simulink model "dc_motor_position_control"  (R2026a)
settings: Solver=VariableStepAuto  StopTime=20  MaxStep=0.01
InitFcn:
  | init_motor;
undefined symbols (not defined in the file or in its folder): ctrl, motor, sensor
libraries: slpidlib x1, simulink x1
settings Model: Creator=seman  LastModifiedBy=seman

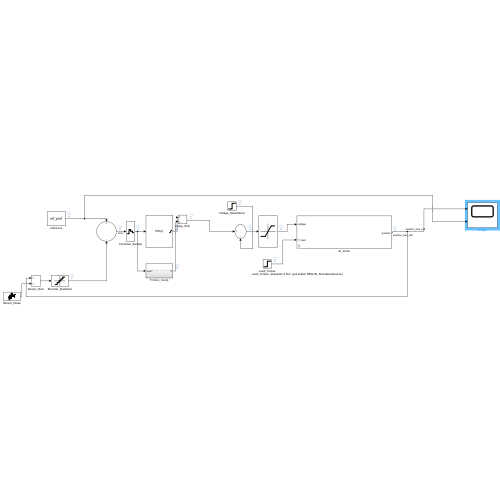
[thumbnail: Simulink's stored preview of the top-level diagram]
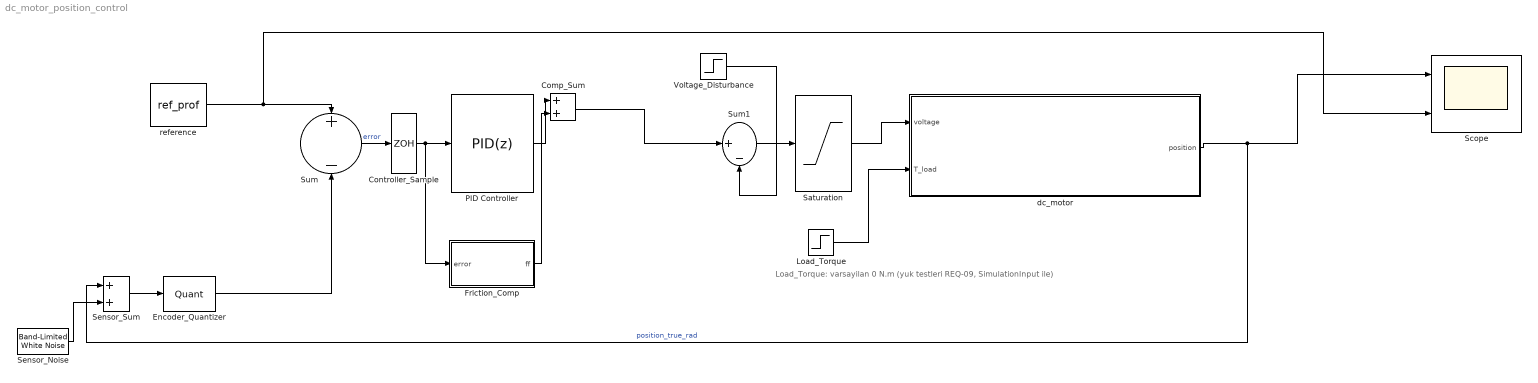
== system dc_motor_position_control ==
  note: Load_Torque: varsayilan 0 N.m (yuk testleri REQ-09, SimulationInput ile)
  Comp_Sum : Sum
  Controller_Sample : ZeroOrderHold  SampleTime=ctrl.Ts
  Encoder_Quantizer : Quantizer  QuantizationInterval=sensor.q_enc
  Friction_Comp : Subsystem
  Load_Torque : Step  Description=Yuk torku girisi (N.m). Varsayilan 0. REQ-09 testleri (run_load_torque_test, run_load_worstcase) basamak yuku SimulationInput ile yalnizca o kosu icin verir.  Time=10  FinalValue=5  SampleTime=0
  PID Controller : slpidlib/PID Controller  Controller=PID  Form=Parallel  TimeDomain=Discrete-time  UseExternalTs=off  SampleTime=ctrl.Ts  IntegratorMethod=Forward Euler  FilterMethod=Backward Euler  ControllerParametersSource=internal  P=ctrl.Kp  I=ctrl.Ki  UseKiTs=off  D=ctrl.Kd  UseExternalDerivativeSource=off  N=ctrl.N  UseFilter=on  TunerSelectOption=Transfer Function Based (PID Tuner App)  InitialConditionSource=internal  InitialConditionForIntegrator=0  InitialConditionForFilter=0  DifferentiatorICPrevScaledInput=0  ExternalReset=none  TrackingMode=off  Kt=1  LimitOutput=on  SatLimitsSource=internal  UpperSaturationLimit=ctrl.Vmax  LowerSaturationLimit=-ctrl.Vmax  LinearizeAsGain=on  AntiWindupMode=back-calculation  Kb=1  LimitIntegrator=off  UpperIntegratorSaturationLimit=inf  LowerIntegratorSaturationLimit=-inf  POutMin=[]  POutMax=[]  IOutMin=[]  IOutMax=[]  DOutMin=[]  DOutMax=[]  NOutMin=[]  NOutMax=[]  SumOutMin=[]  SumOutMax=[]  SaturationOutMin=[]  SaturationOutMax=[]  PParamMin=[]  PParamMax=[]  IParamMin=[]  IParamMax=[]  DParamMin=[]  DParamMax=[]  NParamMin=[]  NParamMax=[]  KbParamMin=[]  KbParamMax=[]  KtParamMin=[]  KtParamMax=[]  KbOutMin=[]  KbOutMax=[]  KtOutMin=[]  KtOutMax=[]  IntegratorOutMin=[]  IntegratorOutMax=[]  FilterOutMin=[]  FilterOutMax=[]  SumI1OutMin=[]  SumI1OutMax=[]  SumI2OutMin=[]  SumI2OutMax=[]  SumI3OutMin=[]  SumI3OutMax=[]  SumI4OutMin=[]  SumI4OutMax=[]  SumDOutMin=[]  SumDOutMax=[]  DifferentiatorOutMin=[]  DifferentiatorOutMax=[]  FilterDiffOutCoefMin=[]  FilterDiffOutCoefMax=[]  ReciprocalOutMin=[]  ReciprocalOutMax=[]  SumDenOutMin=[]  SumDenOutMax=[]  SumNumOutMin=[]  SumNumOutMax=[]  DivideOutMin=[]  DivideOutMax=[]  UdiffTsProdOutMin=[]  UdiffTsProdOutMax=[]  NTsProdOutMin=[]  NTsProdOutMax=[]  UintegralTsProdOutMin=[]  UintegralTsProdOutMax=[]  UngainTsProdOutMin=[]  UngainTsProdOutMax=[]  ClampingZeroOutDataTypeStr=Inherit: Inherit via back propagation  ClampingZeroOutMin=[]  ClampingZeroOutMax=[]  FilterDenConstantOutDataTypeStr=Inherit: Inherit via back propagation  FilterDenConstantOutMin=[]  FilterDenConstantOutMax=[]  PCopyOutDataTypeStr=Inherit: Inherit via back propagation  PCopyOutMin=[]  PCopyOutMax=[]  NCopyOutDataTypeStr=Inherit: Inherit via back propagation  NCopyOutMin=[]  NCopyOutMax=[]  IntegratorContinuousStateAttributes=''  IntegratorStateMustResolveToSignalObject=off  IntegratorRTWStateStorageClass=Auto  FilterContinuousStateAttributes=''  FilterStateMustResolveToSignalObject=off  FilterRTWStateStorageClass=Auto  ParallelPVariant=InternalParameters  IdealPVariant=Disabled  IVariant=InternalParameters  DVariant=InternalParameters  IntegratorVariant=Discrete  SatVariant=Enabled  AWVariant=BackCalculation  PCopyVariant=Disabled  TRVariant=Disabled  FdbkBlocksVariant=Forward  IdealPFdbkVariant=Disabled  SatFdbkVariant=Disabled  DerivativeFilterVariant=BackwardEulerFilter  NVariant=InternalParameters  NCopyVariant=InternalParameters  FilterICVariant=InternalICsFilter  IntegratorICVariant=InternalICs  ExternalResetVariant=Disabled  TRSumVariant=Passthrough  SumFdbkVariant=Disabled  SumVariant=Sum_PID  TsampFilterVariant=InternalTs  TsampNgainVariant=Passthrough  TsampIntegralVariant=Disabled_SignalSpec  ExternalSaturationOutDataTypeStr=Inherit: Same as second input  DerivativeSourceVariant=ErrorSignal  PreIntVariant=InternalPreInt
  Saturation : Saturate  UpperLimit=ctrl.Vmax  LowerLimit=-ctrl.Vmax
  Scope : Scope  NumInputPorts=2
      settings: ActiveDisplayYMinimum=-11.339350762490124  ActiveDisplayYMaximum=102.05415686241113
  Sensor_Noise : simulink/Sources/Band-Limited White Noise  Cov=sensor.noise_cov  Ts=sensor.noise_Ts  seed=[sensor.seed]
  Sensor_Sum : Sum
  Sum : Sum  Inputs=+-
  Sum1 : Sum  Inputs=|+-
  Voltage_Disturbance : Step  Description=Voltaj bozucusu (V). Normalde 0; run_disturbance_test ve run_disturbance_sweep acar.  Time=10  FinalValue=0  SampleTime=0
  dc_motor : Subsystem  InitFcn=""  mask{J=motor.J, B=motor.B, KT=motor.KT, R=motor.R, L=motor.L, KB=motor.KB, Tc=motor.Tc, w_eps=motor.w_eps}
      mask prompts: J "J(KG*M^2)"; B "B(Nm/rad)"; KT "NM/AMPER"; R "R(OHM)"; L "L(H)"; KB "KB(VS/rad)"; Tc "Coulomb surtunme torku (N.m)"; w_eps "Coulomb yumusatma hizi (rad/s)"
  reference : FromWorkspace  Description=Konum referansi (rad). Veri: ref_prof = [zaman konum], init_motor.m icinde. Varsayilan: sabit 50 rad.  VariableName=ref_prof  OutputAfterFinalValue=Holding final value
  wires:
  dc_motor/1(position) -> Scope/1, Sensor_Sum/1  "position_true_rad"
  reference/1 -> Scope/2, Sum/1
  Saturation/1 -> dc_motor/1(voltage)
  Voltage_Disturbance/1 -> Sum1/2
  Sum1/1 -> Saturation/1
  Sensor_Noise/1 -> Sensor_Sum/2
  Sensor_Sum/1 -> Encoder_Quantizer/1
  Encoder_Quantizer/1 -> Sum/2
  Load_Torque/1 -> dc_motor/2(T_load)
  PID Controller/1 -> Comp_Sum/1
  Comp_Sum/1 -> Sum1/1
  Friction_Comp/1(ff) -> Comp_Sum/2
  Sum/1 -> Controller_Sample/1  "error"
  Controller_Sample/1 -> PID Controller/1, Friction_Comp/1(error)

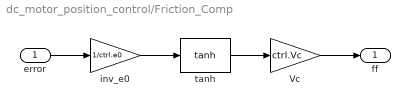
== system dc_motor_position_control/Friction_Comp ==
  error : Inport
  Vc : Gain  Gain=ctrl.Vc
  inv_e0 : Gain  Gain=1/ctrl.e0
  tanh : Trigonometry  Operator=tanh
  ff : Outport
  wires:
  error/1 -> inv_e0/1
  inv_e0/1 -> tanh/1
  tanh/1 -> Vc/1
  Vc/1 -> ff/1

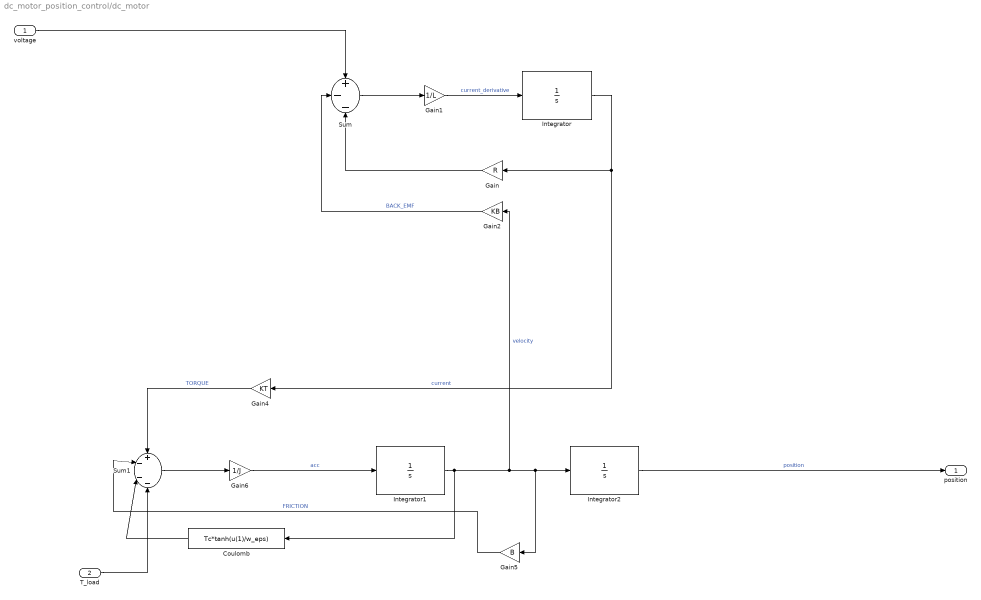
== system dc_motor_position_control/dc_motor ==
  voltage : Inport
  T_load : Inport  Port=2
  Coulomb : Fcn  Expr=Tc*tanh(u(1)/w_eps)
  Gain : Gain  Gain=R
  Gain1 : Gain  Gain=1/L
  Gain2 : Gain  Gain=KB
  Gain4 : Gain  Gain=KT
  Gain5 : Gain  Gain=B
  Gain6 : Gain  Gain=1/J
  Integrator : Integrator
  Integrator1 : Integrator
  Integrator2 : Integrator
  Sum : Sum  Inputs=+--
  Sum1 : Sum  Inputs=+---
  position : Outport
  wires:
  Gain6/1 -> Integrator1/1  "acc"
  Integrator1/1 -> Gain2/1, Integrator2/1, Gain5/1, Coulomb/1  "velocity"
  Gain2/1 -> Sum/2  "BACK_EMF"
  Gain4/1 -> Sum1/1  "TORQUE"
  Integrator/1 -> Gain4/1, Gain/1  "current"
  Gain/1 -> Sum/3
  Sum/1 -> Gain1/1
  Gain1/1 -> Integrator/1  "current_derivative"
  Sum1/1 -> Gain6/1
  Gain5/1 -> Sum1/2  "FRICTION"
  Integrator2/1 -> position/1  "position"
  voltage/1 -> Sum/1
  Coulomb/1 -> Sum1/3
  T_load/1 -> Sum1/4
